simulink model "tvc_pd_educational"  (Simulink 7.0)
settings: Solver=ode45  StartTime=0.0  StopTime=p.attitude_end  MaxStep=0.01  RelTol=1e-8  AbsTol=1e-10
undefined symbols (not defined in the file): p
settings Model: ModelVersion=1.0  ReturnWorkspaceOutputs=on

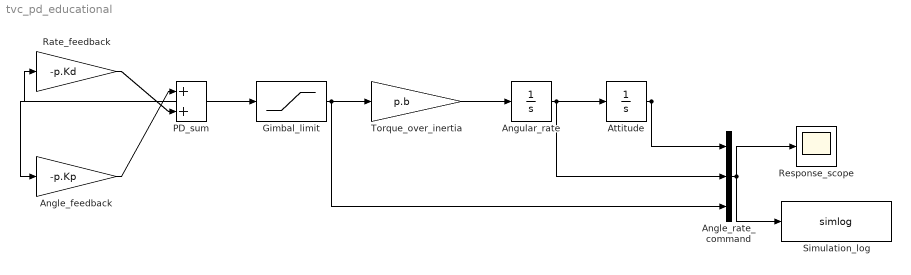
== system tvc_pd_educational ==
  Angle_feedback : Gain  Gain=-p.Kp
  Rate_feedback : Gain  Gain=-p.Kd
  PD_sum : Sum  Inputs=++
  Gimbal_limit : Saturate  UpperLimit=p.delta_max  LowerLimit=-p.delta_max
  Torque_over_inertia : Gain  Gain=p.b
  Angular_rate : Integrator  InitialCondition=p.omega0
  Attitude : Integrator  InitialCondition=p.theta0
  Angle_rate_command : Mux  Inputs=3
  Response_scope : Scope
  Simulation_log : ToWorkspace  VariableName=simlog  SaveFormat=Structure With Time
  wires:
  Angle_feedback/1 -> PD_sum/1
  Rate_feedback/1 -> PD_sum/2
  PD_sum/1 -> Gimbal_limit/1
  Gimbal_limit/1 -> Torque_over_inertia/1, Angle_rate_command/3
  Torque_over_inertia/1 -> Angular_rate/1
  Angular_rate/1 -> Attitude/1, Rate_feedback/1, Angle_rate_command/2
  Attitude/1 -> Angle_feedback/1, Angle_rate_command/1
  Angle_rate_command/1 -> Response_scope/1, Simulation_log/1
